simulink model "HandGuiding_Testbench"  (R2025b)
settings: Solver=FixedStepDiscrete  StartTime=0.0  StopTime=4  FixedStep=0.002  RelTol=1e-3
settings Model: Creator=Compu  LastModifiedBy=Compu

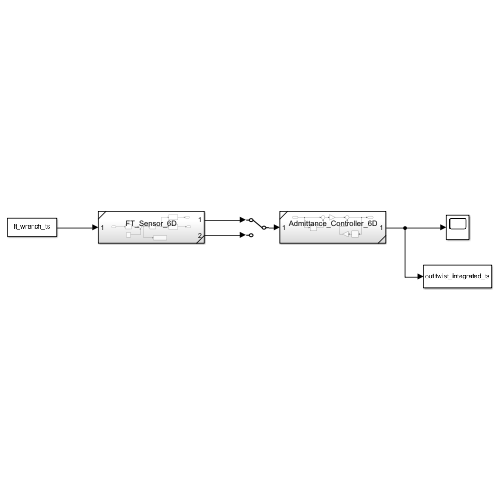
[thumbnail: Simulink's stored preview of the top-level diagram]
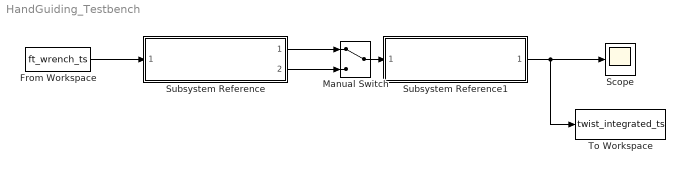
== system HandGuiding_Testbench ==
  From Workspace : FromWorkspace  VariableName=ft_wrench_ts
  Manual Switch : ManualSwitch
  Scope : Scope
      settings: ActiveDisplayYMinimum=-0.030048911817667771  ActiveDisplayYMaximum=0.041575459985877285
  Subsystem Reference : Subsystem  ReferencedSubsystem=FT_Sensor_6D
  Subsystem Reference1 : Subsystem  ReferencedSubsystem=Admittance_Controller_6D
  To Workspace : ToWorkspace  VariableName=twist_integrated_ts  SaveFormat=Timeseries  SampleTime=-1
  wires:
  From Workspace/1 -> Subsystem Reference/1
  Subsystem Reference/1 -> Manual Switch/1
  Subsystem Reference/2 -> Manual Switch/2
  Manual Switch/1 -> Subsystem Reference1/1
  Subsystem Reference1/1 -> Scope/1, To Workspace/1
